simulink library "lib_Grid_AC_Dynamic"  (R2026a)
settings: Solver=VariableStepAuto
undefined symbols (not defined in the file): C_Lines, Cbuses, fref, From_buses, From_nodes, L_Loads, Lines_fromM, Lines_toM, Load_buses, Nbuses, op_Grid_AC_Dynamic, R_Lines, R_Loads, shift_lines, t_close_lines, tap_lines, To_buses, To_nodes
(part 1 of 2)
settings Model: Creator=atomas  LastModifiedBy=atomas

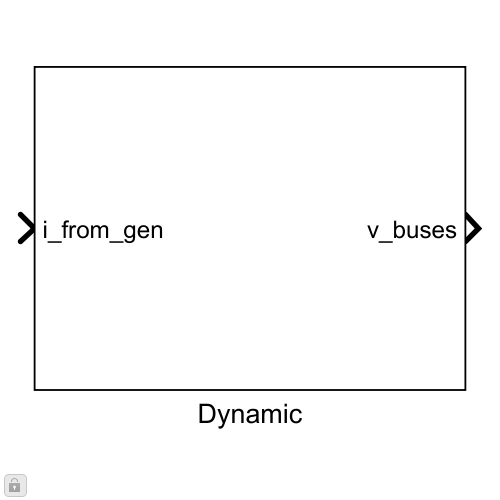
[thumbnail: Simulink's stored preview of the top-level diagram]
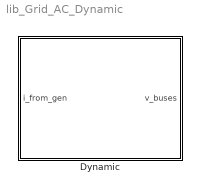
== system lib_Grid_AC_Dynamic ==
  Dynamic : Subsystem  VariantControl=Dynamic

== system lib_Grid_AC_Dynamic/Dynamic ==
  i_from_gen : Inport
  Buses : Subsystem
  Goto Tag Visibility : GotoTagVisibility  GotoTag=Cbuses
  Lines : Subsystem
  Lines to buses : Subsystem
  Loads : Subsystem
  Loads to buses : Subsystem
  Selector2 : Selector  NumberOfDimensions=2  InputPortWidth=Nnodes  IndexOptions=Select all,Index vector (dialog)  Indices=1,Load_buses  OutputSizes=1,1
  Selector4 : Selector  NumberOfDimensions=2  InputPortWidth=Nnodes  IndexOptions=Select all,Index vector (dialog)  Indices=From_nodes,From_buses  OutputSizes=1,1
  Selector6 : Selector  NumberOfDimensions=2  InputPortWidth=Nnodes  IndexOptions=Select all,Index vector (dialog)  Indices=To_nodes,To_buses  OutputSizes=1,1
  Step : Step  Time=t_close_lines  SampleTime=0
  Sum : Sum  Inputs=++|
  Sum1 : Sum  Inputs=|++
  connect : Subsystem
  iCbuses : Subsystem
  iP : Subsystem
  v_buses : Outport
  tag scope: Cbuses=scoped
  wires:
  Buses/1(v) -> [v_buses], v_buses/1
  [i_from_lines] -> Sum/2
  [i_to_loads] -> Sum1/1
  Lines to buses/2(i_out_buses) -> [i_to_lines]
  Loads to buses/1(i_out_buses) -> [i_to_loads]
  iP/1(Out1) -> Loads/3(iP)
  Selector6/1 -> Lines/2(v_out)
  [v_buses] -> Selector2/1
  connect/1(Out1) -> Loads/2(connected)
  [v_buses] -> Selector6/1
  Loads/1(i) -> Loads to buses/1(i_loads)
  Sum/1 -> Buses/1(i_in)
  Selector4/1 -> Lines/1(v_in)
  Selector2/1 -> Loads/1(v_in)
  [v_buses] -> Selector4/1
  [i_to_lines] -> Sum1/2
  Step/1 -> iCbuses/1(In1), Lines/3(connected)
  i_from_gen/1 -> Sum/1
  Sum1/1 -> Buses/2(i_out)
  Lines to buses/1(i_in_buses) -> [i_from_lines]
  Lines/1(i) -> Lines to buses/1(i)
  iCbuses/1(Out1) -> [Cbuses]

== system lib_Grid_AC_Dynamic/Dynamic/Buses ==
  i_in : Inport
  i_out : Inport  Port=2
  Sum : Sum  Inputs=|++++
  dynamic : Subsystem  Variant=on
  only R : Subsystem  Variant=on
  static : Subsystem  Variant=on
  static omega : Subsystem  Variant=on
  v : Outport
  wires:
  only R/1(Out1) -> Sum/4
  i_out/1 -> only R/2(In2), static omega/2(In2), static/2(In2), dynamic/2(In2)
  i_in/1 -> only R/1(In1), static omega/1(In1), static/1(In1), dynamic/1(In1)
  static omega/1(Out1) -> Sum/3
  static/1(Out1) -> Sum/2
  dynamic/1(Out1) -> Sum/1
  Sum/1 -> v/1

== system lib_Grid_AC_Dynamic/Dynamic/Lines ==
  note: tap transformer
  v_in : Inport
  v_out : Inport  Port=2
  connected : Inport  Port=3
  Complex to Real-Imag : ComplexToRealImag
  Constant1 : Constant  Value=zeros(1, length(R_Lines))  VectorParams1D=off
  Gain : Gain  Gain=1./tap_lines.*(cos(shift_lines)-1i*sin(shift_lines))
  Matrix Concatenate : Concatenate  NumInputs=3  Mode=Multidimensional array
  Real-Imag to Complex : RealImagToComplex
  Selector : Selector  NumberOfDimensions=2  InputPortWidth=3  IndexOptions=Index vector (dialog),Select all  Indices=1,1  OutputSizes=1,1
  Selector1 : Selector  NumberOfDimensions=2  InputPortWidth=3  IndexOptions=Index vector (dialog),Select all  Indices=2,1  OutputSizes=1,1
  Sum : Sum  Inputs=|+++
  dynamic : Subsystem  Variant=on
  static : Subsystem  Variant=on
  static omega : Subsystem  Variant=on
  i : Outport
  wires:
  static omega/1(Out1) -> Sum/3
  connected/1 -> static omega/3(In3), static/3(In3), dynamic/3(In3)
  v_out/1 -> static omega/2(In2), static/2(In2), dynamic/2(In2)
  Matrix Concatenate/1 -> static omega/1(In1), static/1(In1), dynamic/1(In1)
  static/1(Out1) -> Sum/2
  dynamic/1(Out1) -> Sum/1
  Sum/1 -> i/1
  v_in/1 -> Selector1/1, Selector/1
  Constant1/1 -> Matrix Concatenate/3
  Complex to Real-Imag/1 -> Matrix Concatenate/1
  Complex to Real-Imag/2 -> Matrix Concatenate/2
  Selector/1 -> Real-Imag to Complex/1
  Selector1/1 -> Real-Imag to Complex/2
  Gain/1 -> Complex to Real-Imag/1
  Real-Imag to Complex/1 -> Gain/1

== system lib_Grid_AC_Dynamic/Dynamic/Lines to buses ==
  i : Inport
  Complex to Real-Imag : ComplexToRealImag
  Constant1 : Constant  Value=zeros(1, length(R_Lines))  VectorParams1D=off
  Gain : Gain  Gain=1./tap_lines.*(cos(shift_lines)-1i*sin(shift_lines))
  Lines_toM : Subsystem  TreatAsAtomicUnit=on
  Matrix Concatenate : Concatenate  NumInputs=3  Mode=Multidimensional array
  Real-Imag to Complex : RealImagToComplex
  Selector : Selector  NumberOfDimensions=2  InputPortWidth=3  IndexOptions=Index vector (dialog),Select all  Indices=1,1  OutputSizes=1,1
  Selector1 : Selector  NumberOfDimensions=2  InputPortWidth=3  IndexOptions=Index vector (dialog),Select all  Indices=2,1  OutputSizes=1,1
  i_in_buses : Outport
  i_out_buses : Outport  Port=2
  wires:
  Lines_toM/2(i_to_lines) -> i_out_buses/1
  i/1 -> Lines_toM/1(i_to), Selector1/1, Selector/1
  Lines_toM/1(i_from_lines) -> i_in_buses/1
  Matrix Concatenate/1 -> Lines_toM/2(i_from)
  Real-Imag to Complex/1 -> Gain/1
  Selector1/1 -> Real-Imag to Complex/2
  Selector/1 -> Real-Imag to Complex/1
  Complex to Real-Imag/1 -> Matrix Concatenate/1
  Complex to Real-Imag/2 -> Matrix Concatenate/2
  Gain/1 -> Complex to Real-Imag/1
  Constant1/1 -> Matrix Concatenate/3

== system lib_Grid_AC_Dynamic/Dynamic/Loads ==
  v_in : Inport
  connected : Inport  Port=2
  iP : Inport  Port=3
  PQ : Subsystem  Variant=on
  Sum : Sum  Inputs=|++++++++
  dynamic PQ : Subsystem  Variant=on
  parallel RL dynamic : Subsystem  Variant=on
  parallel RL static : Subsystem  Variant=on
  parallel RL static omega : Subsystem  Variant=on
  series RL dynamic : Subsystem  Variant=on
  series RL static : Subsystem  Variant=on
  series RL static omega : Subsystem  Variant=on
  i : Outport
  wires:
  parallel RL static omega/1(Out1) -> Sum/8
  connected/1 -> parallel RL static omega/2(In2), parallel RL static/2(In2), parallel RL dynamic/2(In2), dynamic PQ/2(In2), PQ/2(In2), series RL static omega/2(In2), series RL static/1(In1), series RL dynamic/2(In2)
  v_in/1 -> parallel RL static omega/1(In1), parallel RL static/1(In1), parallel RL dynamic/1(In1), dynamic PQ/1(In1), PQ/1(In1), series RL static omega/1(In1), series RL static/2(In2), series RL dynamic/1(In1)
  parallel RL static/1(Out1) -> Sum/7
  parallel RL dynamic/1(Out1) -> Sum/6
  dynamic PQ/1(Out1) -> Sum/5
  iP/1 -> dynamic PQ/3(In3), PQ/3(In3)
  PQ/1(Out1) -> Sum/4
  series RL static omega/1(Out1) -> Sum/3
  series RL static/1(Out1) -> Sum/2
  series RL dynamic/1(Out1) -> Sum/1
  Sum/1 -> i/1

== system lib_Grid_AC_Dynamic/Dynamic/Loads to buses ==
  i_loads : Inport
  LoadsM : Subsystem  TreatAsAtomicUnit=on
  i_out_buses : Outport
  wires:
  i_loads/1 -> LoadsM/1(i)
  LoadsM/1(Out1) -> i_out_buses/1

== system lib_Grid_AC_Dynamic/Dynamic/connect ==
  note: in which load?
      | By default, the max(P)
  Assignment : Assignment  DiagnosticForDimensions=Warning  IndexOptions=Index vector (dialog)  Indices=1  OutputSizes=1
  One3 : Constant  Value=ones(1, length(L_Loads))  VectorParams1D=off  OutDataTypeStr=Inherit: Inherit via back propagation
  Step : Step  InitialValue=1  SampleTime=0
  Out1 : Outport
  wires:
  Assignment/1 -> Out1/1
  One3/1 -> Assignment/1
  Step/1 -> Assignment/2

== system lib_Grid_AC_Dynamic/Dynamic/iCbuses ==
  In1 : Inport
  Constant : Constant  Value=Cbuses  VectorParams1D=off
  Constant1 : Constant  Value=C_Lines  VectorParams1D=off
  Gain : Gain  Gain=1/2
  Saturation : Saturate  UpperLimit=inf  LowerLimit=1e-12
  Subsystem : Subsystem
  Sum3 : Sum  Inputs=|-+
  Switch : Switch  Criteria=u2 > Threshold  SaturateOnIntegerOverflow=off  InputSameDT=off
  Zero : Constant  Value=zeros(1, length(From_buses))  VectorParams1D=off  OutDataTypeStr=Inherit: Inherit via back propagation
  Out1 : Outport
  wires:
  Switch/1 -> Gain/1
  Sum3/1 -> Saturation/1
  Zero/1 -> Switch/1
  Saturation/1 -> Out1/1
  Constant/1 -> Sum3/2
  Gain/1 -> Subsystem/1(In1)
  Constant1/1 -> Switch/3
  In1/1 -> Switch/2
  Subsystem/1(Out1) -> Sum3/1

== system lib_Grid_AC_Dynamic/Dynamic/iP ==
  note: in which load?
      | By default, the max(P)
  Assignment : Assignment  DiagnosticForDimensions=Warning  IndexOptions=Index vector (dialog)  Indices=find(Ploads == max(Ploads), 1)  OutputSizes=1
  Gain : Gain  Gain=0
  One3 : Constant  Value=zeros(1, length(L_Loads))  VectorParams1D=off  OutDataTypeStr=Inherit: Inherit via back propagation
  iP in % : Step  FinalValue=0  SampleTime=0  VectorParams1D=off  ZeroCross=off
  Out1 : Outport
  wires:
  One3/1 -> Assignment/1
  iP in %/1 -> Gain/1
  Assignment/1 -> Out1/1
  Gain/1 -> Assignment/2

== system lib_Grid_AC_Dynamic/Dynamic/Buses/dynamic ==
  note: 1) Add Subsystem or Model blocks as valid variant choices.
      | 2) You cannot connect blocks at this level. At simulation, connectivity is automatically
      | determined, based on the active variant and port name matching.
  In1 : Inport
  In2 : Inport  Port=2
  Active : Subsystem  VariantControl=has_bus_c1 == 1
  Bypass : Subsystem  VariantControl=(default)
  Out1 : Outport

== system lib_Grid_AC_Dynamic/Dynamic/Buses/only R ==
  note: 1) Add Subsystem or Model blocks as valid variant choices.
      | 2) You cannot connect blocks at this level. At simulation, connectivity is automatically
      | determined, based on the active variant and port name matching.
  In1 : Inport
  In2 : Inport  Port=2
  Active : Subsystem  VariantControl=has_bus_c4 == 1
  Bypass : Subsystem  VariantControl=(default)
  Out1 : Outport

== system lib_Grid_AC_Dynamic/Dynamic/Buses/static ==
  note: 1) Add Subsystem or Model blocks as valid variant choices.
      | 2) You cannot connect blocks at this level. At simulation, connectivity is automatically
      | determined, based on the active variant and port name matching.
  In1 : Inport
  In2 : Inport  Port=2
  Active : Subsystem  VariantControl=has_bus_c2 == 1
  Bypass : Subsystem  VariantControl=(default)
  Out1 : Outport

== system lib_Grid_AC_Dynamic/Dynamic/Buses/static omega ==
  note: 1) Add Subsystem or Model blocks as valid variant choices.
      | 2) You cannot connect blocks at this level. At simulation, connectivity is automatically
      | determined, based on the active variant and port name matching.
  In1 : Inport
  In2 : Inport  Port=2
  Active : Subsystem  VariantControl=has_bus_c3 == 1
  Bypass : Subsystem  VariantControl=(default)
  Out1 : Outport

== system lib_Grid_AC_Dynamic/Dynamic/Lines/dynamic ==
  note: 1) Add Subsystem or Model blocks as valid variant choices.
      | 2) You cannot connect blocks at this level. At simulation, connectivity is automatically
      | determined, based on the active variant and port name matching.
  In1 : Inport
  In2 : Inport  Port=2
  In3 : Inport  Port=3
  Active : Subsystem  VariantControl=has_line_c1 == 1
  Bypass : Subsystem  VariantControl=(default)
  Out1 : Outport

== system lib_Grid_AC_Dynamic/Dynamic/Lines/static ==
  note: 1) Add Subsystem or Model blocks as valid variant choices.
      | 2) You cannot connect blocks at this level. At simulation, connectivity is automatically
      | determined, based on the active variant and port name matching.
  In1 : Inport
  In2 : Inport  Port=2
  In3 : Inport  Port=3
  Active : Subsystem  VariantControl=has_line_c2 == 1
  Bypass : Subsystem  VariantControl=(default)
  Out1 : Outport

== system lib_Grid_AC_Dynamic/Dynamic/Lines/static omega ==
  note: 1) Add Subsystem or Model blocks as valid variant choices.
      | 2) You cannot connect blocks at this level. At simulation, connectivity is automatically
      | determined, based on the active variant and port name matching.
  In1 : Inport
  In2 : Inport  Port=2
  In3 : Inport  Port=3
  Active : Subsystem  VariantControl=has_line_c3 == 1
  Bypass : Subsystem  VariantControl=(default)
  Out1 : Outport

== system lib_Grid_AC_Dynamic/Dynamic/Lines to buses/Lines_toM ==
  i_to : Inport  Partition=on  PartitionDimension=1  PartitionWidth=1  PartitionOffset=0
  i_from : Inport  Port=2  Partition=on  PartitionDimension=1  PartitionWidth=1  PartitionOffset=0
  For Each : ForEach  DisableCoverage=on
  State-Space : StateSpace  A=[]  B=[]  C=[]  D=Lines_toM  InitialCondition=0  ParameterTunability=Optimized
  State-Space1 : StateSpace  A=[]  B=[]  C=[]  D=Lines_fromM  InitialCondition=0  ParameterTunability=Optimized
  Transpose{,1..3} (4 alike) : Math  Operator=transpose
  i_from_lines : Outport  ConcatenationDimension=1
  i_to_lines : Outport  Port=2  ConcatenationDimension=1
  wires:
  Transpose1/1 -> i_from_lines/1
  i_to/1 -> Transpose/1
  State-Space/1 -> Transpose1/1
  Transpose/1 -> State-Space/1
  Transpose2/1 -> State-Space1/1
  State-Space1/1 -> Transpose3/1
  i_from/1 -> Transpose2/1
  Transpose3/1 -> i_to_lines/1

== system lib_Grid_AC_Dynamic/Dynamic/Loads/PQ ==
  note: 1) Add Subsystem or Model blocks as valid variant choices.
      | 2) You cannot connect blocks at this level. At simulation, connectivity is automatically
      | determined, based on the active variant and port name matching.
  In1 : Inport
  In2 : Inport  Port=2
  In3 : Inport  Port=3
  Active : Subsystem  VariantControl=has_load_c4 == 1
  Bypass : Subsystem  VariantControl=(default)
  Out1 : Outport

== system lib_Grid_AC_Dynamic/Dynamic/Loads/dynamic PQ ==
  note: 1) Add Subsystem or Model blocks as valid variant choices.
      | 2) You cannot connect blocks at this level. At simulation, connectivity is automatically
      | determined, based on the active variant and port name matching.
  In1 : Inport
  In2 : Inport  Port=2
  In3 : Inport  Port=3
  Active : Subsystem  VariantControl=has_load_c5 == 1
  Bypass : Subsystem  VariantControl=(default)
  Out1 : Outport

== system lib_Grid_AC_Dynamic/Dynamic/Loads/parallel RL dynamic ==
  note: 1) Add Subsystem or Model blocks as valid variant choices.
      | 2) You cannot connect blocks at this level. At simulation, connectivity is automatically
      | determined, based on the active variant and port name matching.
  In1 : Inport
  In2 : Inport  Port=2
  Active : Subsystem  VariantControl=has_load_c6 == 1
  Bypass : Subsystem  VariantControl=(default)
  Out1 : Outport

== system lib_Grid_AC_Dynamic/Dynamic/Loads/parallel RL static ==
  note: 1) Add Subsystem or Model blocks as valid variant choices.
      | 2) You cannot connect blocks at this level. At simulation, connectivity is automatically
      | determined, based on the active variant and port name matching.
  In1 : Inport
  In2 : Inport  Port=2
  Active : Subsystem  VariantControl=has_load_c7 == 1
  Bypass : Subsystem  VariantControl=(default)
  Out1 : Outport

== system lib_Grid_AC_Dynamic/Dynamic/Loads/parallel RL static omega ==
  note: 1) Add Subsystem or Model blocks as valid variant choices.
      | 2) You cannot connect blocks at this level. At simulation, connectivity is automatically
      | determined, based on the active variant and port name matching.
  In1 : Inport
  In2 : Inport  Port=2
  Active : Subsystem  VariantControl=has_load_c8 == 1
  Bypass : Subsystem  VariantControl=(default)
  Out1 : Outport

== system lib_Grid_AC_Dynamic/Dynamic/Loads/series RL dynamic ==
  note: 1) Add Subsystem or Model blocks as valid variant choices.
      | 2) You cannot connect blocks at this level. At simulation, connectivity is automatically
      | determined, based on the active variant and port name matching.
  In1 : Inport
  In2 : Inport  Port=2
  Active : Subsystem  VariantControl=has_load_c1 == 1
  Bypass : Subsystem  VariantControl=(default)
  Out1 : Outport

== system lib_Grid_AC_Dynamic/Dynamic/Loads/series RL static ==
  note: 1) Add Subsystem or Model blocks as valid variant choices.
      | 2) You cannot connect blocks at this level. At simulation, connectivity is automatically
      | determined, based on the active variant and port name matching.
  In1 : Inport
  In2 : Inport  Port=2
  Active : Subsystem  VariantControl=has_load_c2 == 1
  Bypass : Subsystem  VariantControl=(default)
  Out1 : Outport

== system lib_Grid_AC_Dynamic/Dynamic/Loads/series RL static omega ==
  note: 1) Add Subsystem or Model blocks as valid variant choices.
      | 2) You cannot connect blocks at this level. At simulation, connectivity is automatically
      | determined, based on the active variant and port name matching.
  In1 : Inport
  In2 : Inport  Port=2
  Active : Subsystem  VariantControl=has_load_c3 == 1
  Bypass : Subsystem  VariantControl=(default)
  Out1 : Outport

== system lib_Grid_AC_Dynamic/Dynamic/Loads to buses/LoadsM ==
  i : Inport  Partition=on  PartitionDimension=1  PartitionWidth=1  PartitionOffset=0
  Assignment : Assignment  DiagnosticForDimensions=Warning  IndexOptions=Index vector (dialog)  Indices=Load_buses  OutputSizes=1
  For Each : ForEach  DisableCoverage=on
  Zero : Constant  Value=zeros(1,Nbuses)  VectorParams1D=off  OutDataTypeStr=Inherit: Inherit via back propagation
  Out1 : Outport  ConcatenationDimension=1
  wires:
  Assignment/1 -> Out1/1
  i/1 -> Assignment/2
  Zero/1 -> Assignment/1

== system lib_Grid_AC_Dynamic/Dynamic/iCbuses/Subsystem ==
  In1 : Inport
  State-Space : StateSpace  A=[]  B=[]  C=[]  D=Lines_toM  InitialCondition=0  ParameterTunability=Optimized
  State-Space1 : StateSpace  A=[]  B=[]  C=[]  D=Lines_fromM  InitialCondition=0  ParameterTunability=Optimized
  Sum : Sum  Inputs=|++
  Transpose : Math  Operator=transpose
  Transpose1 : Math  Operator=transpose
  Transpose2 : Math  Operator=transpose
  Out1 : Outport
  wires:
  Transpose1/1 -> Sum/1
  State-Space1/1 -> Transpose2/1
  State-Space/1 -> Transpose1/1
  Transpose/1 -> State-Space1/1, State-Space/1
  Sum/1 -> Out1/1
  Transpose2/1 -> Sum/2
  In1/1 -> Transpose/1

== system lib_Grid_AC_Dynamic/Dynamic/Buses/dynamic/Active ==
  In1 : Inport
  In2 : Inport  Port=2
  Impl : Subsystem  VariantControl=dynamic
  Out1 : Outport
  wires:
  Impl/1(v) -> Out1/1
  In2/1 -> Impl/2(i_out)
  In1/1 -> Impl/1(i_in)

== system lib_Grid_AC_Dynamic/Dynamic/Buses/dynamic/Bypass ==
  In1 : Inport
  In2 : Inport  Port=2
  Term1 : Terminator
  Term2 : Terminator
  Zero1 : Constant  Value=zeros(3, Nbuses)  VectorParams1D=off
  Out1 : Outport
  wires:
  Zero1/1 -> Out1/1
  In2/1 -> Term2/1
  In1/1 -> Term1/1

== system lib_Grid_AC_Dynamic/Dynamic/Buses/only R/Active ==
  In1 : Inport
  In2 : Inport  Port=2
  Impl : Subsystem  VariantControl=only R
  Out1 : Outport
  wires:
  Impl/1(v) -> Out1/1
  In2/1 -> Impl/2(i_out)
  In1/1 -> Impl/1(i_in)

== system lib_Grid_AC_Dynamic/Dynamic/Buses/only R/Bypass ==
  In1 : Inport
  In2 : Inport  Port=2
  Term1 : Terminator
  Term2 : Terminator
  Zero1 : Constant  Value=zeros(3, Nbuses)  VectorParams1D=off
  Out1 : Outport
  wires:
  Zero1/1 -> Out1/1
  In2/1 -> Term2/1
  In1/1 -> Term1/1

== system lib_Grid_AC_Dynamic/Dynamic/Buses/static/Active ==
  In1 : Inport
  In2 : Inport  Port=2
  Impl : Subsystem  VariantControl=static
  Out1 : Outport
  wires:
  Impl/1(v) -> Out1/1
  In2/1 -> Impl/2(i_out)
  In1/1 -> Impl/1(i_in)

== system lib_Grid_AC_Dynamic/Dynamic/Buses/static/Bypass ==
  In1 : Inport
  In2 : Inport  Port=2
  Term1 : Terminator
  Term2 : Terminator
  Zero1 : Constant  Value=zeros(3, Nbuses)  VectorParams1D=off
  Out1 : Outport
  wires:
  Zero1/1 -> Out1/1
  In2/1 -> Term2/1
  In1/1 -> Term1/1

== system lib_Grid_AC_Dynamic/Dynamic/Buses/static omega/Active ==
  In1 : Inport
  In2 : Inport  Port=2
  Impl : Subsystem  VariantControl=static omega
  Out1 : Outport
  wires:
  Impl/1(v) -> Out1/1
  In2/1 -> Impl/2(i_out)
  In1/1 -> Impl/1(i_in)

== system lib_Grid_AC_Dynamic/Dynamic/Buses/static omega/Bypass ==
  In1 : Inport
  In2 : Inport  Port=2
  Term1 : Terminator
  Term2 : Terminator
  Zero1 : Constant  Value=zeros(3, Nbuses)  VectorParams1D=off
  Out1 : Outport
  wires:
  Zero1/1 -> Out1/1
  In2/1 -> Term2/1
  In1/1 -> Term1/1

== system lib_Grid_AC_Dynamic/Dynamic/Lines/dynamic/Active ==
  In1 : Inport
  In2 : Inport  Port=2
  In3 : Inport  Port=3
  Impl : Subsystem  VariantControl=dynamic
  Out1 : Outport
  wires:
  Impl/1(i) -> Out1/1
  In3/1 -> Impl/3(connected)
  In2/1 -> Impl/2(v_out)
  In1/1 -> Impl/1(v_in_d)

== system lib_Grid_AC_Dynamic/Dynamic/Lines/dynamic/Bypass ==
  In1 : Inport
  In2 : Inport  Port=2
  In3 : Inport  Port=3
  Term1 : Terminator
  Term2 : Terminator
  Term3 : Terminator
  Zero1 : Constant  Value=zeros(3, max(1, length(From_buses)))  VectorParams1D=off
  Out1 : Outport
  wires:
  Zero1/1 -> Out1/1
  In3/1 -> Term3/1
  In2/1 -> Term2/1
  In1/1 -> Term1/1

== system lib_Grid_AC_Dynamic/Dynamic/Lines/static/Active ==
  In1 : Inport
  In2 : Inport  Port=2
  In3 : Inport  Port=3
  Impl : Subsystem  VariantControl=static
  Out1 : Outport
  wires:
  Impl/1(i) -> Out1/1
  In3/1 -> Impl/3(connected)
  In2/1 -> Impl/2(v_out_d)
  In1/1 -> Impl/1(v_in)

== system lib_Grid_AC_Dynamic/Dynamic/Lines/static/Bypass ==
  In1 : Inport
  In2 : Inport  Port=2
  In3 : Inport  Port=3
  Term1 : Terminator
  Term2 : Terminator
  Term3 : Terminator
  Zero1 : Constant  Value=zeros(3, max(1, length(From_buses)))  VectorParams1D=off
  Out1 : Outport
  wires:
  Zero1/1 -> Out1/1
  In3/1 -> Term3/1
  In2/1 -> Term2/1
  In1/1 -> Term1/1

== system lib_Grid_AC_Dynamic/Dynamic/Lines/static omega/Active ==
  In1 : Inport
  In2 : Inport  Port=2
  In3 : Inport  Port=3
  Impl : Subsystem  VariantControl=static_omega
  Out1 : Outport
  wires:
  Impl/1(i) -> Out1/1
  In3/1 -> Impl/3(connected)
  In2/1 -> Impl/2(v_out)
  In1/1 -> Impl/1(v_in_d)

== system lib_Grid_AC_Dynamic/Dynamic/Lines/static omega/Bypass ==
  In1 : Inport
  In2 : Inport  Port=2
  In3 : Inport  Port=3
  Term1 : Terminator
  Term2 : Terminator
  Term3 : Terminator
  Zero1 : Constant  Value=zeros(3, max(1, length(From_buses)))  VectorParams1D=off
  Out1 : Outport
  wires:
  Zero1/1 -> Out1/1
  In3/1 -> Term3/1
  In2/1 -> Term2/1
  In1/1 -> Term1/1

== system lib_Grid_AC_Dynamic/Dynamic/Loads/PQ/Active ==
  In1 : Inport
  In2 : Inport  Port=2
  In3 : Inport  Port=3
  Impl : Subsystem  VariantControl=PQ
  Out1 : Outport
  wires:
  Impl/1(i) -> Out1/1
  In3/1 -> Impl/3(iP)
  In2/1 -> Impl/2(connected)
  In1/1 -> Impl/1(v_in)

== system lib_Grid_AC_Dynamic/Dynamic/Loads/PQ/Bypass ==
  In1 : Inport
  In2 : Inport  Port=2
  In3 : Inport  Port=3
  Term1 : Terminator
  Term2 : Terminator
  Term3 : Terminator
  Zero1 : Constant  Value=zeros(3, max(1, length(L_Loads)))  VectorParams1D=off
  Out1 : Outport
  wires:
  Zero1/1 -> Out1/1
  In3/1 -> Term3/1
  In2/1 -> Term2/1
  In1/1 -> Term1/1

== system lib_Grid_AC_Dynamic/Dynamic/Loads/dynamic PQ/Active ==
  In1 : Inport
  In2 : Inport  Port=2
  In3 : Inport  Port=3
  Impl : Subsystem  VariantControl=dynamic_PQ
  Out1 : Outport
  wires:
  Impl/1(i) -> Out1/1
  In3/1 -> Impl/3(iP)
  In2/1 -> Impl/2(connected)
  In1/1 -> Impl/1(v_in)

== system lib_Grid_AC_Dynamic/Dynamic/Loads/dynamic PQ/Bypass ==
  In1 : Inport
  In2 : Inport  Port=2
  In3 : Inport  Port=3
  Term1 : Terminator
  Term2 : Terminator
  Term3 : Terminator
  Zero1 : Constant  Value=zeros(3, max(1, length(L_Loads)))  VectorParams1D=off
  Out1 : Outport
  wires:
  Zero1/1 -> Out1/1
  In3/1 -> Term3/1
  In2/1 -> Term2/1
  In1/1 -> Term1/1

== system lib_Grid_AC_Dynamic/Dynamic/Loads/parallel RL dynamic/Active ==
  In1 : Inport
  In2 : Inport  Port=2
  Impl : Subsystem  VariantControl=dynamic
  Out1 : Outport
  wires:
  Impl/1(i) -> Out1/1
  In2/1 -> Impl/2(connected)
  In1/1 -> Impl/1(v_in)

== system lib_Grid_AC_Dynamic/Dynamic/Loads/parallel RL dynamic/Bypass ==
  In1 : Inport
  In2 : Inport  Port=2
  Term1 : Terminator
  Term2 : Terminator
  Zero1 : Constant  Value=zeros(3, max(1, length(L_Loads)))  VectorParams1D=off
  Out1 : Outport
  wires:
  Zero1/1 -> Out1/1
  In2/1 -> Term2/1
  In1/1 -> Term1/1

== system lib_Grid_AC_Dynamic/Dynamic/Loads/parallel RL static/Active ==
  In1 : Inport
  In2 : Inport  Port=2
  Impl : Subsystem  VariantControl=dynamic
  Out1 : Outport
  wires:
  Impl/1(i) -> Out1/1
  In2/1 -> Impl/2(connected)
  In1/1 -> Impl/1(v_in)

== system lib_Grid_AC_Dynamic/Dynamic/Loads/parallel RL static/Bypass ==
  In1 : Inport
  In2 : Inport  Port=2
  Term1 : Terminator
  Term2 : Terminator
  Zero1 : Constant  Value=zeros(3, max(1, length(L_Loads)))  VectorParams1D=off
  Out1 : Outport
  wires:
  Zero1/1 -> Out1/1
  In2/1 -> Term2/1
  In1/1 -> Term1/1

== system lib_Grid_AC_Dynamic/Dynamic/Loads/parallel RL static omega/Active ==
  In1 : Inport
  In2 : Inport  Port=2
  Impl : Subsystem  VariantControl=dynamic
  Out1 : Outport
  wires:
  Impl/1(i) -> Out1/1
  In2/1 -> Impl/2(connected)
  In1/1 -> Impl/1(v_in)

== system lib_Grid_AC_Dynamic/Dynamic/Loads/parallel RL static omega/Bypass ==
  In1 : Inport
  In2 : Inport  Port=2
  Term1 : Terminator
  Term2 : Terminator
  Zero1 : Constant  Value=zeros(3, max(1, length(L_Loads)))  VectorParams1D=off
  Out1 : Outport
  wires:
  Zero1/1 -> Out1/1
  In2/1 -> Term2/1
  In1/1 -> Term1/1

== system lib_Grid_AC_Dynamic/Dynamic/Loads/series RL dynamic/Active ==
  In1 : Inport
  In2 : Inport  Port=2
  Impl : Subsystem  VariantControl=dynamic
  Out1 : Outport
  wires:
  Impl/1(i) -> Out1/1
  In2/1 -> Impl/2(connected)
  In1/1 -> Impl/1(v_in)

== system lib_Grid_AC_Dynamic/Dynamic/Loads/series RL dynamic/Bypass ==
  In1 : Inport
  In2 : Inport  Port=2
  Term1 : Terminator
  Term2 : Terminator
  Zero1 : Constant  Value=zeros(3, max(1, length(L_Loads)))  VectorParams1D=off
  Out1 : Outport
  wires:
  Zero1/1 -> Out1/1
  In2/1 -> Term2/1
  In1/1 -> Term1/1

== system lib_Grid_AC_Dynamic/Dynamic/Loads/series RL static/Active ==
  In1 : Inport
  In2 : Inport  Port=2
  Impl : Subsystem  VariantControl=static
  Out1 : Outport
  wires:
  Impl/1(i) -> Out1/1
  In2/1 -> Impl/2(v_in)
  In1/1 -> Impl/1(connected)

== system lib_Grid_AC_Dynamic/Dynamic/Loads/series RL static/Bypass ==
  In1 : Inport
  In2 : Inport  Port=2
  Term1 : Terminator
  Term2 : Terminator
  Zero1 : Constant  Value=zeros(3, max(1, length(L_Loads)))  VectorParams1D=off
  Out1 : Outport
  wires:
  Zero1/1 -> Out1/1
  In2/1 -> Term2/1
  In1/1 -> Term1/1

== system lib_Grid_AC_Dynamic/Dynamic/Loads/series RL static omega/Active ==
  In1 : Inport
  In2 : Inport  Port=2
  Impl : Subsystem  VariantControl=static_omega
  Out1 : Outport
  wires:
  Impl/1(i) -> Out1/1
  In2/1 -> Impl/2(connected)
  In1/1 -> Impl/1(v_in)

== system lib_Grid_AC_Dynamic/Dynamic/Loads/series RL static omega/Bypass ==
  In1 : Inport
  In2 : Inport  Port=2
  Term1 : Terminator
  Term2 : Terminator
  Zero1 : Constant  Value=zeros(3, max(1, length(L_Loads)))  VectorParams1D=off
  Out1 : Outport
  wires:
  Zero1/1 -> Out1/1
  In2/1 -> Term2/1
  In1/1 -> Term1/1

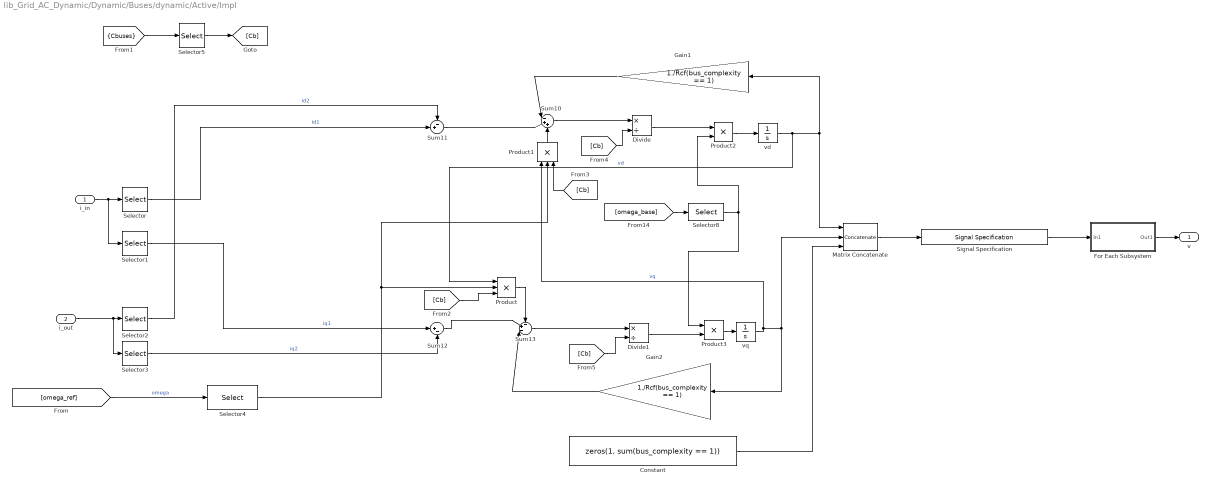
== system lib_Grid_AC_Dynamic/Dynamic/Buses/dynamic/Active/Impl ==
  i_in : Inport
  i_out : Inport  Port=2
  Constant : Constant  Value=zeros(1, sum(bus_complexity == 1))  VectorParams1D=off
  Divide : Product  Inputs=*/
  Divide1 : Product  Inputs=*/
  For Each Subsystem : Subsystem  TreatAsAtomicUnit=on
  Gain1 : Gain  Gain=1./Rcf(bus_complexity == 1)
  Gain2 : Gain  Gain=1./Rcf(bus_complexity == 1)
  Matrix Concatenate : Concatenate  NumInputs=3  Mode=Multidimensional array
  Product : Product  Inputs=3
  Product1 : Product  Inputs=3
  Product2 : Product
  Product3 : Product
  Selector : Selector  NumberOfDimensions=2  InputPortWidth=3  IndexOptions=Index vector (dialog),Index vector (dialog)  Indices=1,find(bus_complexity == 1)  OutputSizes=1,1
  Selector1 : Selector  NumberOfDimensions=2  InputPortWidth=3  IndexOptions=Index vector (dialog),Index vector (dialog)  Indices=2,find(bus_complexity == 1)  OutputSizes=1,1
  Selector2 : Selector  NumberOfDimensions=2  InputPortWidth=3  IndexOptions=Index vector (dialog),Index vector (dialog)  Indices=1,find(bus_complexity == 1)  OutputSizes=1,1
  Selector3 : Selector  NumberOfDimensions=2  InputPortWidth=3  IndexOptions=Index vector (dialog),Index vector (dialog)  Indices=2,find(bus_complexity == 1)  OutputSizes=1,1
  Selector4 : Selector  InputPortWidth=length(fref.ref_units)  IndexOptions=Index vector (dialog)  Indices=fref.buses(bus_complexity == 1)  OutputSizes=1
  Selector5 : Selector  InputPortWidth=length(Cbuses)  IndexOptions=Index vector (dialog)  Indices=find(bus_complexity == 1)  OutputSizes=1
  Selector8 : Selector  InputPortWidth=length(fref.ref_units)  IndexOptions=Index vector (dialog)  Indices=fref.buses(bus_complexity == 1)  OutputSizes=1
  Signal Specification : SignalSpecification  Dimensions=[3 sum(bus_complexity == 1)]
  Sum10 : Sum  Inputs=|-++
  Sum11 : Sum  Inputs=-+|
  Sum12 : Sum  Inputs=|+-
  Sum13 : Sum  Inputs=-+-|
  vd : Integrator  InitialCondition=op_Grid_AC_Dynamic.Buses_dynamic_Active_Impl_vd
  vq : Integrator  InitialCondition=op_Grid_AC_Dynamic.Buses_dynamic_Active_Impl_vq
  v : Outport
  wires:
  Sum13/1 -> Divide1/1
  [Cb] -> Divide1/2
  [Cb] -> Divide/2
  [Cb] -> Product1/3
  [Cb] -> Product/3
  Selector5/1 -> [Cb]
  [Cbuses] -> Selector5/1
  Product3/1 -> vq/1
  Product2/1 -> vd/1
  Selector8/1 -> Product3/1, Product2/2
  [omega_base] -> Selector8/1
  Divide1/1 -> Product3/2
  Divide/1 -> Product2/1
  Selector4/1 -> Product/2, Product1/2
  Constant/1 -> Matrix Concatenate/3
  Signal Specification/1 -> For Each Subsystem/1(In1)
  For Each Subsystem/1(Out1) -> v/1
  Matrix Concatenate/1 -> Signal Specification/1
  i_out/1 -> Selector2/1, Selector3/1
  i_in/1 -> Selector1/1, Selector/1
  Selector3/1 -> Sum12/2  "iq2"
  Selector1/1 -> Sum12/1  "iq1"
  Selector2/1 -> Sum11/1  "id2"
  Selector/1 -> Sum11/2  "id1"
  vd/1 -> Product/1, Matrix Concatenate/1, Gain1/1  "vd"
  Sum12/1 -> Sum13/2
  Gain1/1 -> Sum10/1
  [omega_ref] -> Selector4/1  "omega"
  Sum11/1 -> Sum10/2
  Product/1 -> Sum13/1
  Gain2/1 -> Sum13/3
  Product1/1 -> Sum10/3
  vq/1 -> Matrix Concatenate/2, Gain2/1, Product1/1  "vq"
  Sum10/1 -> Divide/1

== system lib_Grid_AC_Dynamic/Dynamic/Buses/only R/Active/Impl ==
  i_in : Inport
  i_out : Inport  Port=2
  Constant : Constant  Value=zeros(1, sum(bus_complexity == 4))  VectorParams1D=off
  For Each Subsystem : Subsystem  TreatAsAtomicUnit=on
  Gain : Gain  Gain=Rcf(bus_complexity == 4)
  Gain2 : Gain  Gain=Rcf(bus_complexity == 4)
  Matrix Concatenate : Concatenate  NumInputs=3  Mode=Multidimensional array
  Selector : Selector  NumberOfDimensions=2  InputPortWidth=3  IndexOptions=Index vector (dialog),Index vector (dialog)  Indices=1,find(bus_complexity == 4)  OutputSizes=1,1
  Selector1 : Selector  NumberOfDimensions=2  InputPortWidth=3  IndexOptions=Index vector (dialog),Index vector (dialog)  Indices=2,find(bus_complexity == 4)  OutputSizes=1,1
  Selector2 : Selector  NumberOfDimensions=2  InputPortWidth=3  IndexOptions=Index vector (dialog),Index vector (dialog)  Indices=1,find(bus_complexity == 4)  OutputSizes=1,1
  Selector3 : Selector  NumberOfDimensions=2  InputPortWidth=3  IndexOptions=Index vector (dialog),Index vector (dialog)  Indices=2,find(bus_complexity == 4)  OutputSizes=1,1
  Sum1 : Sum  Inputs=|+-
  Sum2 : Sum  Inputs=|+-
  v : Outport
  wires:
  Constant/1 -> Matrix Concatenate/3
  For Each Subsystem/1(Out1) -> v/1
  i_out/1 -> Selector3/1, Selector2/1
  Matrix Concatenate/1 -> For Each Subsystem/1(In1)
  i_in/1 -> Selector1/1, Selector/1
  Gain/1 -> Matrix Concatenate/1
  Gain2/1 -> Matrix Concatenate/2
  Selector2/1 -> Sum1/2
  Selector/1 -> Sum1/1  "id"
  Selector3/1 -> Sum2/2  "iq2"
  Sum2/1 -> Gain2/1  "iq"
  Sum1/1 -> Gain/1  "id"
  Selector1/1 -> Sum2/1  "iq1"

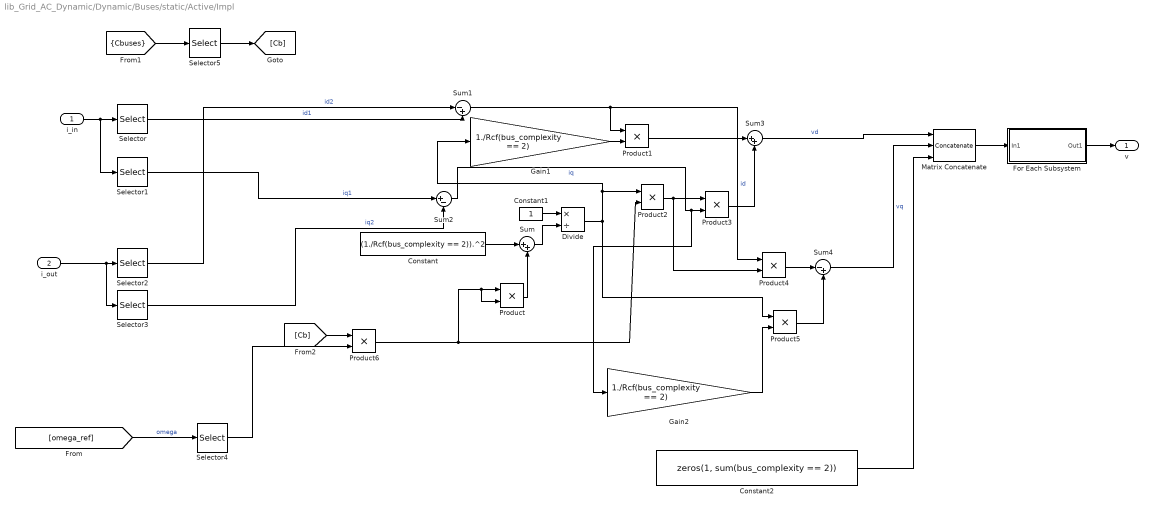
== system lib_Grid_AC_Dynamic/Dynamic/Buses/static/Active/Impl ==
  i_in : Inport
  i_out : Inport  Port=2
  Constant : Constant  Value=(1./Rcf(bus_complexity == 2)).^2  VectorParams1D=off
  Constant1 : Constant
  Constant2 : Constant  Value=zeros(1, sum(bus_complexity == 2))  VectorParams1D=off
  Divide : Product  Inputs=*/
  For Each Subsystem : Subsystem  TreatAsAtomicUnit=on
  Gain1 : Gain  Gain=1./Rcf(bus_complexity == 2)
  Gain2 : Gain  Gain=1./Rcf(bus_complexity == 2)
  Matrix Concatenate : Concatenate  NumInputs=3  Mode=Multidimensional array
  Product{,1..6} (7 alike) : Product
  Selector : Selector  NumberOfDimensions=2  InputPortWidth=3  IndexOptions=Index vector (dialog),Index vector (dialog)  Indices=1,find(bus_complexity == 2)  OutputSizes=1,1
  Selector1 : Selector  NumberOfDimensions=2  InputPortWidth=3  IndexOptions=Index vector (dialog),Index vector (dialog)  Indices=2,find(bus_complexity == 2)  OutputSizes=1,1
  Selector2 : Selector  NumberOfDimensions=2  InputPortWidth=3  IndexOptions=Index vector (dialog),Index vector (dialog)  Indices=1,find(bus_complexity == 2)  OutputSizes=1,1
  Selector3 : Selector  NumberOfDimensions=2  InputPortWidth=3  IndexOptions=Index vector (dialog),Index vector (dialog)  Indices=2,find(bus_complexity == 2)  OutputSizes=1,1
  Selector4 : Selector  InputPortWidth=length(fref.ref_units)  IndexOptions=Index vector (dialog)  Indices=fref.buses(bus_complexity == 2)  OutputSizes=1
  Selector5 : Selector  InputPortWidth=length(Cbuses)  IndexOptions=Index vector (dialog)  Indices=find(bus_complexity == 2)  OutputSizes=1
  Sum : Sum  Inputs=|++
  Sum1 : Sum  Inputs=|-+
  Sum2 : Sum  Inputs=|+-
  Sum3 : Sum  Inputs=|++
  Sum4 : Sum  Inputs=|-+
  v : Outport
  wires:
  [Cb] -> Product6/1
  [Cbuses] -> Selector5/1
  Selector5/1 -> [Cb]
  Selector4/1 -> Product6/2
  Constant2/1 -> Matrix Concatenate/3
  For Each Subsystem/1(Out1) -> v/1
  i_out/1 -> Selector3/1, Selector2/1
  Matrix Concatenate/1 -> For Each Subsystem/1(In1)
  i_in/1 -> Selector1/1, Selector/1
  Selector3/1 -> Sum2/2  "iq2"
  Selector1/1 -> Sum2/1  "iq1"
  Selector2/1 -> Sum1/1  "id2"
  Selector/1 -> Sum1/2  "id1"
  [omega_ref] -> Selector4/1  "omega"
  Sum3/1 -> Matrix Concatenate/1  "vd"
  Sum4/1 -> Matrix Concatenate/2  "vq"
  Constant/1 -> Sum/1
  Sum/1 -> Divide/2
  Product6/1 -> Product2/2, Product/2, Product/1
  Product/1 -> Sum/2
  Constant1/1 -> Divide/1
  Sum1/1 -> Product1/1, Product4/1  "id"
  Sum2/1 -> Gain2/1, Product3/2  "iq"
  Gain1/1 -> Product1/2
  Divide/1 -> Product5/1, Gain1/1, Product2/1
  Product1/1 -> Sum3/1
  Product3/1 -> Sum3/2
  Product2/1 -> Product4/2, Product3/1
  Product4/1 -> Sum4/1
  Gain2/1 -> Product5/2
  Product5/1 -> Sum4/2

== system lib_Grid_AC_Dynamic/Dynamic/Buses/static omega/Active/Impl ==
  i_in : Inport
  i_out : Inport  Port=2
  Constant : Constant  Value=zeros(1, sum(bus_complexity == 3))  VectorParams1D=off
  For Each Subsystem : Subsystem  TreatAsAtomicUnit=on
  Gain : Gain  Gain=1./((1./Rcf(bus_complexity == 3)).^2+Cbuses(bus_complexity == 3).^2)
  Gain1 : Gain  Gain=1./((1./Rcf(bus_complexity == 3)).^2+Cbuses(bus_complexity == 3).^2)
  Gain3 : Gain  Gain=1./Rcf(bus_complexity == 3)
  Gain5 : Gain  Gain=1./Rcf(bus_complexity == 3)
  IC : InitialCondition  Value=op_Grid_AC_Dynamic.bus_static_omega_ic
  LPF : Subsystem  Commented=through
  Matrix Concatenate : Concatenate  NumInputs=3  Mode=Multidimensional array
  Product : Product
  Product1 : Product
  Selector : Selector  NumberOfDimensions=2  InputPortWidth=3  IndexOptions=Index vector (dialog),Index vector (dialog)  Indices=1,find(bus_complexity == 3)  OutputSizes=1,1
  Selector1 : Selector  NumberOfDimensions=2  InputPortWidth=3  IndexOptions=Index vector (dialog),Index vector (dialog)  Indices=2,find(bus_complexity == 3)  OutputSizes=1,1
  Selector2 : Selector  NumberOfDimensions=2  InputPortWidth=3  IndexOptions=Index vector (dialog),Index vector (dialog)  Indices=1,find(bus_complexity == 3)  OutputSizes=1,1
  Selector3 : Selector  NumberOfDimensions=2  InputPortWidth=3  IndexOptions=Index vector (dialog),Index vector (dialog)  Indices=2,find(bus_complexity == 3)  OutputSizes=1,1
  Selector5 : Selector  InputPortWidth=length(Cbuses)  IndexOptions=Index vector (dialog)  Indices=find(bus_complexity == 3)  OutputSizes=1
  Sum : Sum  Inputs=|++
  Sum1 : Sum  Inputs=|+-
  Sum2 : Sum  Inputs=|+-
  Sum4 : Sum  Inputs=|-+
  v : Outport
  wires:
  [Cb] -> Product1/2
  [Cb] -> Product/2
  [Cbuses] -> Selector5/1
  Selector5/1 -> [Cb]
  IC/1 -> For Each Subsystem/1(In1)
  LPF/1(out) -> IC/1
  Matrix Concatenate/1 -> LPF/1(in)
  Constant/1 -> Matrix Concatenate/3
  For Each Subsystem/1(Out1) -> v/1
  i_out/1 -> Selector2/1, Selector3/1
  i_in/1 -> Selector/1, Selector1/1
  Sum/1 -> Matrix Concatenate/1
  Sum4/1 -> Matrix Concatenate/2
  Gain5/1 -> Sum4/2
  Product/1 -> Sum4/1
  Product1/1 -> Sum/2
  Gain3/1 -> Sum/1
  Gain1/1 -> Gain5/1, Product1/1
  Gain/1 -> Gain3/1, Product/1
  Selector2/1 -> Sum1/2
  Selector/1 -> Sum1/1  "id"
  Selector3/1 -> Sum2/2  "iq2"
  Sum2/1 -> Gain1/1  "iq"
  Sum1/1 -> Gain/1  "id"
  Selector1/1 -> Sum2/1  "iq1"

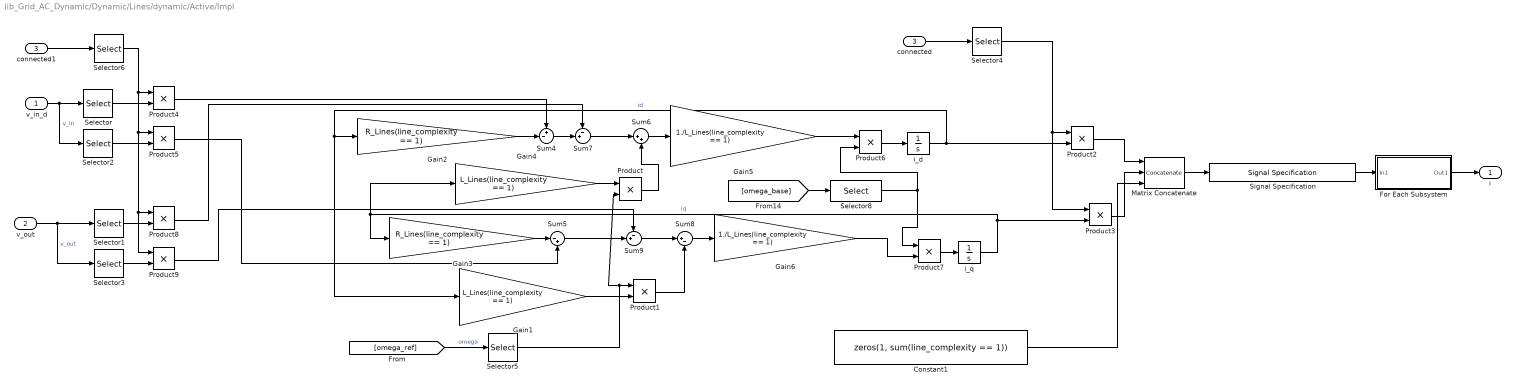
== system lib_Grid_AC_Dynamic/Dynamic/Lines/dynamic/Active/Impl ==
  v_in_d : Inport
  v_out : Inport  Port=2
  connected : Inport  Port=3
  Constant1 : Constant  Value=zeros(1, sum(line_complexity == 1))  VectorParams1D=off
  For Each Subsystem : Subsystem  TreatAsAtomicUnit=on
  Gain1 : Gain  Gain=L_Lines(line_complexity == 1)
  Gain2 : Gain  Gain=R_Lines(line_complexity == 1)
  Gain3 : Gain  Gain=R_Lines(line_complexity == 1)
  Gain4 : Gain  Gain=L_Lines(line_complexity == 1)
  Gain5 : Gain  Gain=1./L_Lines(line_complexity == 1)
  Gain6 : Gain  Gain=1./L_Lines(line_complexity == 1)
  Matrix Concatenate : Concatenate  NumInputs=3  Mode=Multidimensional array
  Product{,1..9} (10 alike) : Product
  Selector : Selector  NumberOfDimensions=2  InputPortWidth=3  IndexOptions=Index vector (dialog),Index vector (dialog)  Indices=1,find(line_complexity == 1)  OutputSizes=1,1
  Selector1 : Selector  NumberOfDimensions=2  InputPortWidth=3  IndexOptions=Index vector (dialog),Index vector (dialog)  Indices=1,find(line_complexity == 1)  OutputSizes=1,1
  Selector2 : Selector  NumberOfDimensions=2  InputPortWidth=3  IndexOptions=Index vector (dialog),Index vector (dialog)  Indices=2,find(line_complexity == 1)  OutputSizes=1,1
  Selector3 : Selector  NumberOfDimensions=2  InputPortWidth=3  IndexOptions=Index vector (dialog),Index vector (dialog)  Indices=2,find(line_complexity == 1)  OutputSizes=1,1
  Selector4 : Selector  InputPortWidth=length(From_buses)  IndexOptions=Index vector (dialog)  Indices=find(line_complexity == 1)  OutputSizes=1
  Selector5 : Selector  InputPortWidth=length(fref.ref_units)  IndexOptions=Index vector (dialog)  Indices=fref.lines(line_complexity == 1)  OutputSizes=1
  Selector6 : Selector  InputPortWidth=length(From_buses)  IndexOptions=Index vector (dialog)  Indices=find(line_complexity == 1)  OutputSizes=1
  Selector8 : Selector  InputPortWidth=length(fref.ref_units)  IndexOptions=Index vector (dialog)  Indices=fref.lines(line_complexity == 1)  OutputSizes=1
  Signal Specification : SignalSpecification  Dimensions=[3 sum(line_complexity == 1)]
  Sum4 : Sum  Inputs=+-|
  Sum5 : Sum  Inputs=|-+
  Sum6 : Sum  Inputs=|++
  Sum7 : Sum  Inputs=-+|
  Sum8 : Sum  Inputs=|+-
  Sum9 : Sum  Inputs=-+|
  connected1 : InportShadow  Port=3
  i_d : Integrator  InitialCondition=op_Grid_AC_Dynamic.Lines_dynamic_Active_Impl_i_d
  i_q : Integrator  InitialCondition=op_Grid_AC_Dynamic.Lines_dynamic_Active_Impl_i_q
  i : Outport
  wires:
  Selector3/1 -> Product9/2
  Selector1/1 -> Product8/2
  Selector2/1 -> Product5/2
  Selector6/1 -> Product4/1, Product5/1, Product8/1, Product9/1
  Selector/1 -> Product4/2
  connected1/1 -> Selector6/1
  Product7/1 -> i_q/1
  Product6/1 -> i_d/1
  Gain6/1 -> Product7/2
  Gain5/1 -> Product6/1
  [omega_base] -> Selector8/1
  Selector8/1 -> Product7/1, Product6/2
  Selector5/1 -> Product1/1, Product/2
  Constant1/1 -> Matrix Concatenate/3
  Signal Specification/1 -> For Each Subsystem/1(In1)
  For Each Subsystem/1(Out1) -> i/1
  Selector4/1 -> Product2/1, Product3/1
  Product9/1 -> Sum9/1
  Product8/1 -> Sum7/1
  Product4/1 -> Sum4/1
  Product3/1 -> Matrix Concatenate/2
  Product2/1 -> Matrix Concatenate/1
  Matrix Concatenate/1 -> Signal Specification/1
  connected/1 -> Selector4/1
  Product5/1 -> Sum5/2
  v_in_d/1 -> Selector/1, Selector2/1  "v_in"
  Gain2/1 -> Sum4/2
  i_d/1 -> Product2/2, Gain2/1, Gain1/1  "id"
  Sum6/1 -> Gain5/1
  [omega_ref] -> Selector5/1  "omega"
  Product/1 -> Sum6/2
  Sum8/1 -> Gain6/1
  Sum4/1 -> Sum7/2
  Product1/1 -> Sum8/2
  Gain4/1 -> Product/1
  Sum7/1 -> Sum6/1
  Gain3/1 -> Sum5/1
  Sum5/1 -> Sum9/2
  i_q/1 -> Product3/2, Gain4/1, Gain3/1  "iq"
  Gain1/1 -> Product1/2
  Sum9/1 -> Sum8/1
  v_out/1 -> Selector1/1, Selector3/1  "v_out"

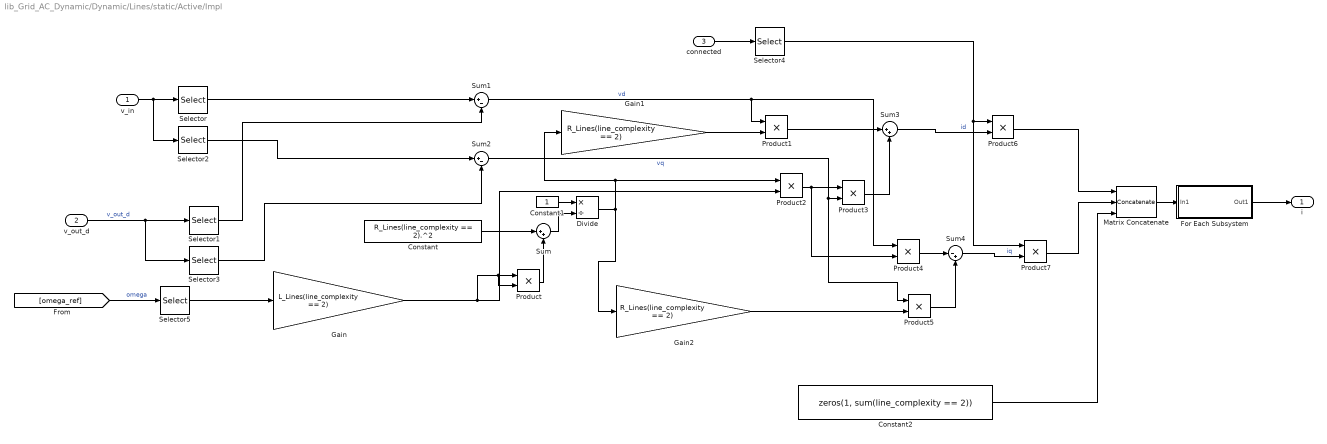
== system lib_Grid_AC_Dynamic/Dynamic/Lines/static/Active/Impl ==
  v_in : Inport
  v_out_d : Inport  Port=2
  connected : Inport  Port=3
  Constant : Constant  Value=R_Lines(line_complexity == 2).^2  VectorParams1D=off
  Constant1 : Constant
  Constant2 : Constant  Value=zeros(1, sum(line_complexity == 2))  VectorParams1D=off
  Divide : Product  Inputs=*/
  For Each Subsystem : Subsystem  TreatAsAtomicUnit=on
  Gain : Gain  Gain=L_Lines(line_complexity == 2)
  Gain1 : Gain  Gain=R_Lines(line_complexity == 2)
  Gain2 : Gain  Gain=R_Lines(line_complexity == 2)
  Matrix Concatenate : Concatenate  NumInputs=3  Mode=Multidimensional array
  Product{,1..7} (8 alike) : Product
  Selector : Selector  NumberOfDimensions=2  InputPortWidth=3  IndexOptions=Index vector (dialog),Index vector (dialog)  Indices=1,find(line_complexity == 2)  OutputSizes=1,1
  Selector1 : Selector  NumberOfDimensions=2  InputPortWidth=3  IndexOptions=Index vector (dialog),Index vector (dialog)  Indices=1,find(line_complexity == 2)  OutputSizes=1,1
  Selector2 : Selector  NumberOfDimensions=2  InputPortWidth=3  IndexOptions=Index vector (dialog),Index vector (dialog)  Indices=2,find(line_complexity == 2)  OutputSizes=1,1
  Selector3 : Selector  NumberOfDimensions=2  InputPortWidth=3  IndexOptions=Index vector (dialog),Index vector (dialog)  Indices=2,find(line_complexity == 2)  OutputSizes=1,1
  Selector4 : Selector  InputPortWidth=length(From_buses)  IndexOptions=Index vector (dialog)  Indices=find(line_complexity == 2)  OutputSizes=1
  Selector5 : Selector  InputPortWidth=length(fref.ref_units)  IndexOptions=Index vector (dialog)  Indices=fref.lines(line_complexity == 2)  OutputSizes=1
  Sum : Sum  Inputs=|++
  Sum1 : Sum  Inputs=|+-
  Sum2 : Sum  Inputs=|+-
  Sum3 : Sum  Inputs=|++
  Sum4 : Sum  Inputs=|-+
  i : Outport
  wires:
  Selector5/1 -> Gain/1
  Constant2/1 -> Matrix Concatenate/3
  For Each Subsystem/1(Out1) -> i/1
  Selector4/1 -> Product6/1, Product7/1
  Product7/1 -> Matrix Concatenate/2
  Product6/1 -> Matrix Concatenate/1
  Matrix Concatenate/1 -> For Each Subsystem/1(In1)
  Selector/1 -> Sum1/1
  Selector2/1 -> Sum2/1
  Selector3/1 -> Sum2/2
  Selector1/1 -> Sum1/2
  connected/1 -> Selector4/1
  v_in/1 -> Selector/1, Selector2/1
  v_out_d/1 -> Selector1/1, Selector3/1  "v_out_d"
  Sum/1 -> Divide/2
  Gain2/1 -> Product5/2
  Product/1 -> Sum/2
  Product1/1 -> Sum3/1
  Product5/1 -> Sum4/2
  Constant/1 -> Sum/1
  Sum2/1 -> Product3/2, Product5/1  "vq"
  Gain/1 -> Product/1, Product/2, Product2/2
  Constant1/1 -> Divide/1
  Product3/1 -> Sum3/2
  Sum1/1 -> Product4/1, Product1/1  "vd"
  Divide/1 -> Product2/1, Gain1/1, Gain2/1
  Product4/1 -> Sum4/1
  Product2/1 -> Product3/1, Product4/2
  Gain1/1 -> Product1/2
  Sum3/1 -> Product6/2  "id"
  Sum4/1 -> Product7/2  "iq"
  [omega_ref] -> Selector5/1  "omega"

== system lib_Grid_AC_Dynamic/Dynamic/Lines/static omega/Active/Impl ==
  v_in_d : Inport
  v_out : Inport  Port=2
  connected : Inport  Port=3
  Constant1 : Constant  Value=zeros(1, sum(line_complexity == 3))  VectorParams1D=off
  For Each Subsystem : Subsystem  TreatAsAtomicUnit=on
  Gain : Gain  Gain=1./(R_Lines(line_complexity == 3).^2+L_Lines(line_complexity == 3).^2)
  Gain1 : Gain  Gain=1./(R_Lines(line_complexity == 3).^2+L_Lines(line_complexity == 3).^2)
  Gain3 : Gain  Gain=R_Lines(line_complexity == 3)
  Gain4 : Gain  Gain=L_Lines(line_complexity == 3)
  Gain5 : Gain  Gain=L_Lines(line_complexity == 3)
  Gain6 : Gain  Gain=R_Lines(line_complexity == 3)
  Matrix Concatenate : Concatenate  NumInputs=3  Mode=Multidimensional array
  Product2 : Product
  Product3 : Product
  Selector : Selector  NumberOfDimensions=2  InputPortWidth=3  IndexOptions=Index vector (dialog),Index vector (dialog)  Indices=1,find(line_complexity == 3)  OutputSizes=1,1
  Selector1 : Selector  NumberOfDimensions=2  InputPortWidth=3  IndexOptions=Index vector (dialog),Index vector (dialog)  Indices=1,find(line_complexity == 3)  OutputSizes=1,1
  Selector2 : Selector  NumberOfDimensions=2  InputPortWidth=3  IndexOptions=Index vector (dialog),Index vector (dialog)  Indices=2,find(line_complexity == 3)  OutputSizes=1,1
  Selector3 : Selector  NumberOfDimensions=2  InputPortWidth=3  IndexOptions=Index vector (dialog),Index vector (dialog)  Indices=2,find(line_complexity == 3)  OutputSizes=1,1
  Selector4 : Selector  InputPortWidth=length(From_buses)  IndexOptions=Index vector (dialog)  Indices=find(line_complexity == 3)  OutputSizes=1
  Sum : Sum  Inputs=|++
  Sum1 : Sum  Inputs=|+-
  Sum2 : Sum  Inputs=|+-
  Sum3 : Sum  Inputs=|-+
  i : Outport
  wires:
  Constant1/1 -> Matrix Concatenate/3
  For Each Subsystem/1(Out1) -> i/1
  Selector4/1 -> Product2/1, Product3/1
  Selector1/1 -> Sum1/2
  v_out/1 -> Selector1/1, Selector3/1
  Selector2/1 -> Sum2/1
  Selector/1 -> Sum1/1
  v_in_d/1 -> Selector/1, Selector2/1  "v_in"
  Product3/1 -> Matrix Concatenate/2
  Product2/1 -> Matrix Concatenate/1
  Matrix Concatenate/1 -> For Each Subsystem/1(In1)
  connected/1 -> Selector4/1
  Gain6/1 -> Sum3/2
  Sum3/1 -> Product3/2
  Gain5/1 -> Sum3/1
  Sum/1 -> Product2/2
  Gain1/1 -> Gain6/1, Gain4/1
  Gain4/1 -> Sum/2
  Gain3/1 -> Sum/1
  Gain/1 -> Gain5/1, Gain3/1
  Sum2/1 -> Gain1/1  "vq"
  Sum1/1 -> Gain/1  "vd"
  Selector3/1 -> Sum2/2  "v_out_q"

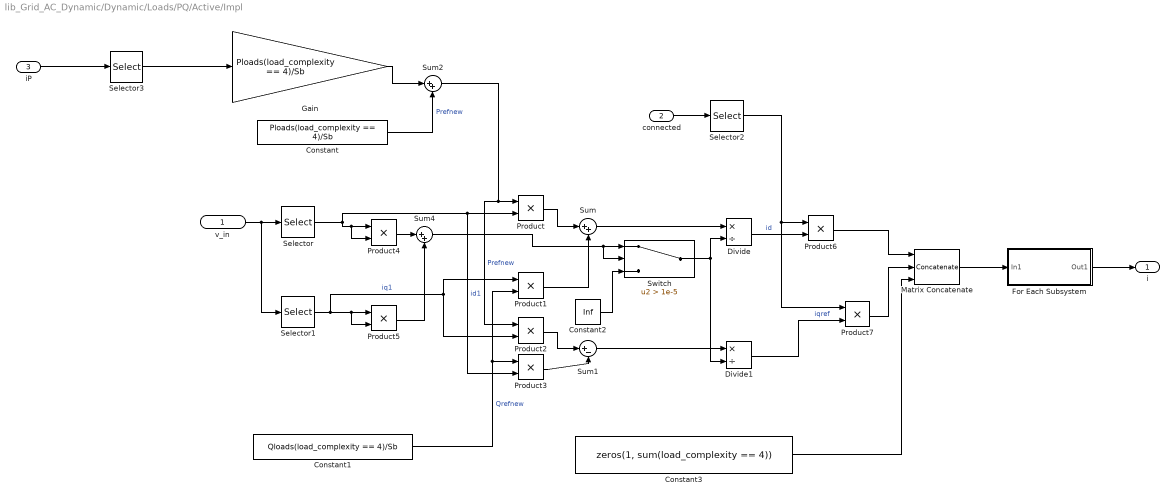
== system lib_Grid_AC_Dynamic/Dynamic/Loads/PQ/Active/Impl ==
  v_in : Inport
  connected : Inport  Port=2
  iP : Inport  Port=3
  Constant : Constant  Value=Ploads(load_complexity == 4)/Sb  VectorParams1D=off
  Constant1 : Constant  Value=Qloads(load_complexity == 4)/Sb  VectorParams1D=off
  Constant2 : Constant  Value=Inf
  Constant3 : Constant  Value=zeros(1, sum(load_complexity == 4))  VectorParams1D=off
  Divide : Product  Inputs=*/
  Divide1 : Product  Inputs=*/
  For Each Subsystem : Subsystem  TreatAsAtomicUnit=on
  Gain : Gain  Gain=Ploads(load_complexity == 4)/Sb
  Matrix Concatenate : Concatenate  NumInputs=3  Mode=Multidimensional array
  Product{,1..7} (8 alike) : Product
  Selector : Selector  NumberOfDimensions=2  InputPortWidth=3  IndexOptions=Index vector (dialog),Index vector (dialog)  Indices=1,find(load_complexity == 4)  OutputSizes=1,1
  Selector1 : Selector  NumberOfDimensions=2  InputPortWidth=3  IndexOptions=Index vector (dialog),Index vector (dialog)  Indices=2,find(load_complexity == 4)  OutputSizes=1,1
  Selector2 : Selector  InputPortWidth=length(R_Loads)  IndexOptions=Index vector (dialog)  Indices=find(load_complexity == 4)  OutputSizes=1
  Selector3 : Selector  InputPortWidth=length(R_Loads)  IndexOptions=Index vector (dialog)  Indices=find(load_complexity == 4)  OutputSizes=1
  Sum : Sum  Inputs=|++
  Sum1 : Sum  Inputs=|+-
  Sum2 : Sum  Inputs=|++
  Sum4 : Sum  Inputs=|++
  Switch : Switch  Criteria=u2 > Threshold  Threshold=1e-5  ZeroCross=off  SaturateOnIntegerOverflow=off  InputSameDT=off
  i : Outport
  wires:
  Constant/1 -> Sum2/2  "Prefnew"
  iP/1 -> Selector3/1
  Gain/1 -> Sum2/1
  Selector3/1 -> Gain/1
  Constant3/1 -> Matrix Concatenate/3
  For Each Subsystem/1(Out1) -> i/1
  Selector2/1 -> Product7/1, Product6/1
  Product7/1 -> Matrix Concatenate/2
  Product6/1 -> Matrix Concatenate/1
  Matrix Concatenate/1 -> For Each Subsystem/1(In1)
  Selector1/1 -> Product1/1, Product2/2, Product5/2, Product5/1  "iq1"
  Selector/1 -> Product3/2, Product/2, Product4/2, Product4/1  "id1"
  Divide1/1 -> Product7/2  "iqref"
  Divide/1 -> Product6/2  "id"
  connected/1 -> Selector2/1
  Sum1/1 -> Divide1/1
  Constant2/1 -> Switch/3
  Sum4/1 -> Switch/2, Switch/1
  Switch/1 -> Divide/2, Divide1/2
  Sum/1 -> Divide/1
  Product4/1 -> Sum4/1
  Constant1/1 -> Product1/2, Product3/1  "Qrefnew"
  Product5/1 -> Sum4/2
  Product3/1 -> Sum1/2
  v_in/1 -> Selector/1, Selector1/1
  Product2/1 -> Sum1/1
  Sum2/1 -> Product2/1, Product/1  "Prefnew"
  Product/1 -> Sum/1
  Product1/1 -> Sum/2
